simulink model "quad_sim"  (R2024b)
settings: Solver=ode4  StartTime=0.0  StopTime=qsim.StopTime  FixedStep=qsim.dt  RelTol=1e-3
PreLoadFcn:
  | if ~exist('qsim','var') || ~exist('quad','var') || ~exist('ideal','var') || ~exist('CtrlIn','var'), run(fullfile(fileparts(which('quad_sim_params')),'quad_sim_params.m')); end
values from neighbouring files (symbols this model uses):
  qsim = quad_sim_derive(qsim, quad)    [quad_scenario.m]    (also in quad_sim_params.m = quad_scenario(qsim, quad, ideal, 'hover'))
  quad = evalin('base', 'quad')    [run_quad_scenarios.m]
libraries: aerolibprivatev1p5 x1
Description:
  | Model 1: 5" quad 6-DOF plant + controller slot (Variant Subsystem "Controller", qsim.ctrl: 1 ideal, 2 board_fast, 3 board_circuit). Run quad_sim_params first.
settings Model: Creator=doubi  LastModifiedBy=doubi
settings DataIOCC: SaveOutput=off  SaveTime=off
settings DebuggingCC: AlgebraicLoopMsg=error

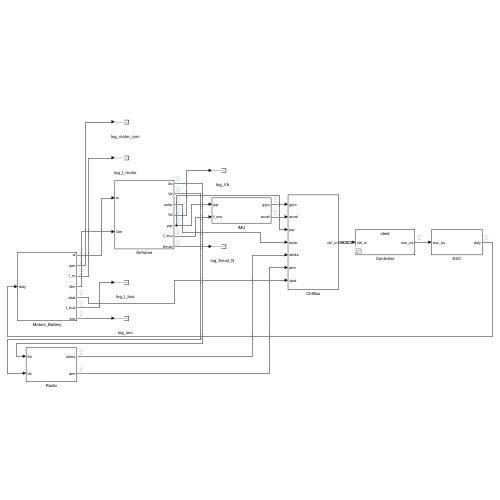
[thumbnail: Simulink's stored preview of the top-level diagram]
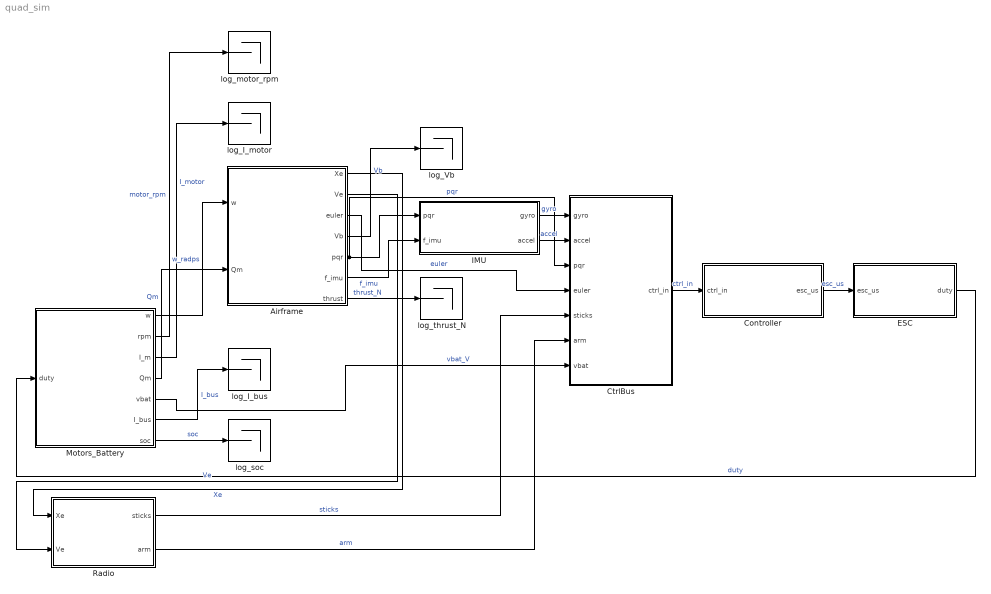
== system quad_sim ==
  Airframe : Subsystem
  Controller : Subsystem  Description=Controller slot. qsim.ctrl selects: 1 ideal (ctrl_ideal.slx), 2 board_fast, 3 board_circuit (sim/pid_board/pid_board.slx). Interface = Inport ctrl_in (bus CtrlIn), Outport esc_us [4x1] double us.  Variant=on
  CtrlBus : Subsystem
  ESC : Subsystem
  IMU : Subsystem
  Motors_Battery : Subsystem
  Radio : Subsystem
  log_I_bus : Terminator
  log_I_motor : Terminator
  log_Vb : Terminator
  log_motor_rpm : Terminator
  log_soc : Terminator
  log_thrust_N : Terminator
  wires:
  IMU/2(accel) -> CtrlBus/2(accel)  "accel"
  Motors_Battery/1(w) -> Airframe/1(w)  "w_radps"
  Motors_Battery/6(I_bus) -> log_I_bus/1  "I_bus"
  Motors_Battery/2(rpm) -> log_motor_rpm/1  "motor_rpm"
  Motors_Battery/7(soc) -> log_soc/1  "soc"
  Motors_Battery/3(I_m) -> log_I_motor/1  "I_motor"
  Motors_Battery/4(Qm) -> Airframe/2(Qm)  "Qm"
  Radio/1(sticks) -> CtrlBus/5(sticks)  "sticks"
  Motors_Battery/5(vbat) -> CtrlBus/7(vbat)  "vbat_V"
  Radio/2(arm) -> CtrlBus/6(arm)  "arm"
  Airframe/1(Xe) -> Radio/1(Xe)  "Xe"
  Airframe/2(Ve) -> Radio/2(Ve)  "Ve"
  Airframe/3(euler) -> CtrlBus/4(euler)  "euler"
  Airframe/4(Vb) -> log_Vb/1  "Vb"
  Airframe/5(pqr) -> IMU/1(pqr), CtrlBus/3(pqr)  "pqr"
  Airframe/6(f_imu) -> IMU/2(f_imu)  "f_imu"
  Airframe/7(thrust) -> log_thrust_N/1  "thrust_N"
  IMU/1(gyro) -> CtrlBus/1(gyro)  "gyro"
  CtrlBus/1(ctrl_in) -> Controller/1(ctrl_in)  "ctrl_in"
  Controller/1(esc_us) -> ESC/1(esc_us)  "esc_us"
  ESC/1(duty) -> Motors_Battery/1(duty)  "duty"

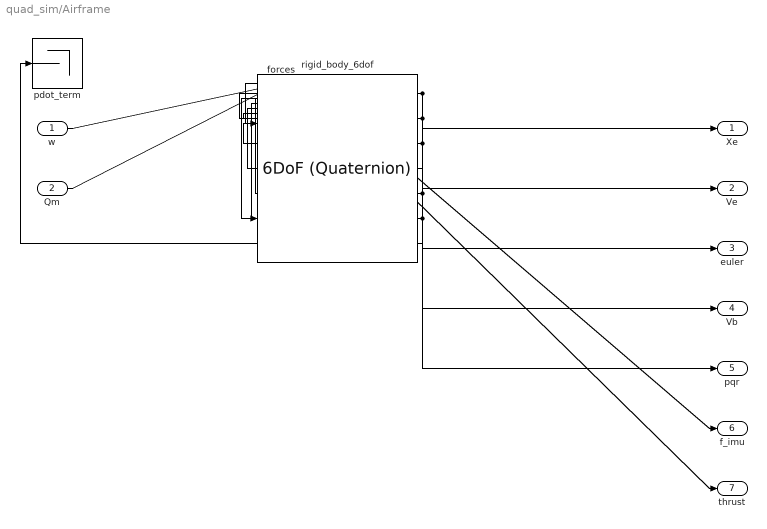
== system quad_sim/Airframe ==
  w : Inport
  Qm : Inport  Port=2
  forces : MATLAB Function  TreatAsAtomicUnit=on  mask{P=qsim.p}
  pdot_term : Terminator
  rigid_body_6dof : aerolibprivatev1p5/6DoF (Quaternion)  xme_0=qsim.init.Xe0  Vm_0=[0 0 0]  eul_0=[0 0 0]  pm_0=[0 0 0]  Mass=quad.mass.total  Inertia=quad.inertia.J  k_quat=1.0
  Xe : Outport
  Ve : Outport  Port=2
  euler : Outport  Port=3
  Vb : Outport  Port=4
  pqr : Outport  Port=5
  f_imu : Outport  Port=6
  thrust : Outport  Port=7
  wires:
  w/1 -> forces/1(w)
  Qm/1 -> forces/2(Qm)
  rigid_body_6dof/5 -> forces/3(Vb), Vb/1
  rigid_body_6dof/6 -> forces/4(wb), pqr/1
  rigid_body_6dof/4 -> forces/5(DCM)
  rigid_body_6dof/2 -> forces/6(Xe), Xe/1
  rigid_body_6dof/1 -> forces/7(Ve), Ve/1
  rigid_body_6dof/3 -> forces/8(eul), euler/1
  forces/1(F_b) -> rigid_body_6dof/1
  forces/2(M_b) -> rigid_body_6dof/2
  rigid_body_6dof/7 -> pdot_term/1
  forces/3(f_imu) -> f_imu/1
  forces/4(T) -> thrust/1

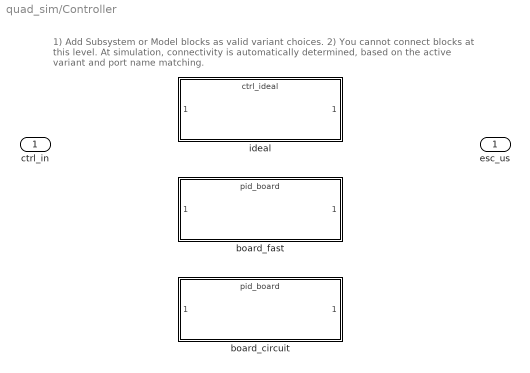
== system quad_sim/Controller ==
  note: 1) Add Subsystem or Model blocks as valid variant choices.
      | 2) You cannot connect blocks at this level. At simulation, connectivity is automatically
      | determined, based on the active variant and port name matching.
  ctrl_in : Inport
  board_circuit : ModelReference  ModelNameDialog=pid_board  ParameterArgumentNames=board_variant  ParameterArgumentValues=2  UsingDefaultArgumentValue=0  SimulationMode=Normal  VariantControl=qsim.ctrl == 3  ModelReferenceVersion=1.1
  board_fast : ModelReference  ModelNameDialog=pid_board  ParameterArgumentNames=board_variant  ParameterArgumentValues=1  UsingDefaultArgumentValue=0  SimulationMode=Normal  VariantControl=qsim.ctrl == 2  ModelReferenceVersion=1.1
  ideal : ModelReference  ModelNameDialog=ctrl_ideal  SimulationMode=Normal  VariantControl=qsim.ctrl == 1  ModelReferenceVersion=1.1
  esc_us : Outport

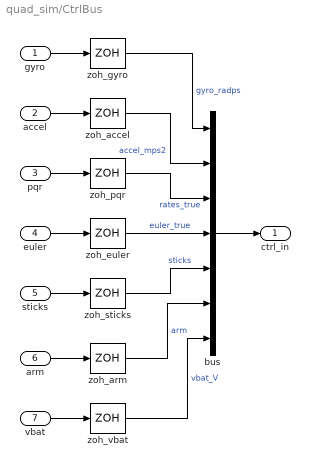
== system quad_sim/CtrlBus ==
  gyro : Inport
  accel : Inport  Port=2
  pqr : Inport  Port=3
  euler : Inport  Port=4
  sticks : Inport  Port=5
  arm : Inport  Port=6
  vbat : Inport  Port=7
  bus : BusCreator  Inputs=7  OutDataTypeStr=Bus: CtrlIn  NonVirtualBus=on
  zoh_accel : ZeroOrderHold  SampleTime=qsim.Ts_bus
  zoh_arm : ZeroOrderHold  SampleTime=qsim.Ts_bus
  zoh_euler : ZeroOrderHold  SampleTime=qsim.Ts_bus
  zoh_gyro : ZeroOrderHold  SampleTime=qsim.Ts_bus
  zoh_pqr : ZeroOrderHold  SampleTime=qsim.Ts_bus
  zoh_sticks : ZeroOrderHold  SampleTime=qsim.Ts_bus
  zoh_vbat : ZeroOrderHold  SampleTime=qsim.Ts_bus
  ctrl_in : Outport
  wires:
  sticks/1 -> zoh_sticks/1
  gyro/1 -> zoh_gyro/1
  zoh_gyro/1 -> bus/1  "gyro_radps"
  vbat/1 -> zoh_vbat/1
  arm/1 -> zoh_arm/1
  accel/1 -> zoh_accel/1
  pqr/1 -> zoh_pqr/1
  euler/1 -> zoh_euler/1
  zoh_accel/1 -> bus/2  "accel_mps2"
  zoh_pqr/1 -> bus/3  "rates_true"
  zoh_euler/1 -> bus/4  "euler_true"
  zoh_sticks/1 -> bus/5  "sticks"
  zoh_arm/1 -> bus/6  "arm"
  zoh_vbat/1 -> bus/7  "vbat_V"
  bus/1 -> ctrl_in/1

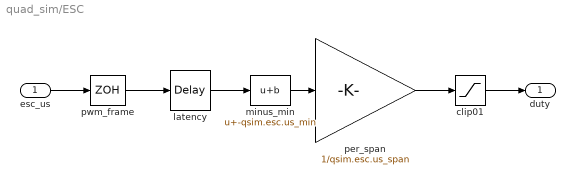
== system quad_sim/ESC ==
  esc_us : Inport
  clip01 : Saturate  UpperLimit=1  LowerLimit=0
  latency : TransportDelay  DelayTime=qsim.esc.delay  InitialOutput=qsim.esc.us0  BufferSize=4096
  minus_min : Bias  Bias=-qsim.esc.us_min  SaturateOnIntegerOverflow=off
  per_span : Gain  Gain=1/qsim.esc.us_span
  pwm_frame : ZeroOrderHold  SampleTime=qsim.esc.Ts
  duty : Outport
  wires:
  minus_min/1 -> per_span/1
  esc_us/1 -> pwm_frame/1
  pwm_frame/1 -> latency/1
  latency/1 -> minus_min/1
  per_span/1 -> clip01/1
  clip01/1 -> duty/1

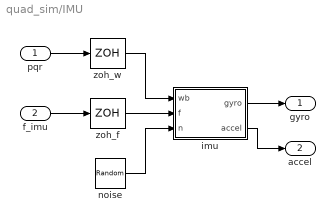
== system quad_sim/IMU ==
  pqr : Inport
  f_imu : Inport  Port=2
  imu : MATLAB Function  TreatAsAtomicUnit=on  mask{P=qsim.imu}
  noise : RandomNumber  Seed=qsim.imu.seed  SampleTime=qsim.imu.Ts
  zoh_f : ZeroOrderHold  SampleTime=qsim.imu.Ts
  zoh_w : ZeroOrderHold  SampleTime=qsim.imu.Ts
  gyro : Outport
  accel : Outport  Port=2
  wires:
  imu/2(accel) -> accel/1
  zoh_f/1 -> imu/2(f)
  pqr/1 -> zoh_w/1
  f_imu/1 -> zoh_f/1
  zoh_w/1 -> imu/1(wb)
  imu/1(gyro) -> gyro/1
  noise/1 -> imu/3(n)

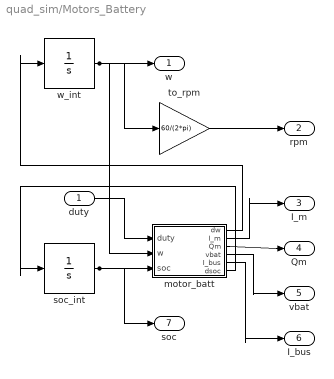
== system quad_sim/Motors_Battery ==
  duty : Inport
  motor_batt : MATLAB Function  TreatAsAtomicUnit=on  mask{P=qsim.p}
  soc_int : Integrator  InitialCondition=qsim.init.soc0  LimitOutput=on  UpperSaturationLimit=1  LowerSaturationLimit=0
  to_rpm : Gain  Gain=60/(2*pi)
  w_int : Integrator  InitialCondition=qsim.init.w0  LimitOutput=on  LowerSaturationLimit=0
  w : Outport
  rpm : Outport  Port=2
  I_m : Outport  Port=3
  Qm : Outport  Port=4
  vbat : Outport  Port=5
  I_bus : Outport  Port=6
  soc : Outport  Port=7
  wires:
  w_int/1 -> motor_batt/2(w), w/1, to_rpm/1
  to_rpm/1 -> rpm/1
  motor_batt/4(vbat) -> vbat/1
  duty/1 -> motor_batt/1(duty)
  soc_int/1 -> motor_batt/3(soc), soc/1
  motor_batt/1(dw) -> w_int/1
  motor_batt/2(I_m) -> I_m/1
  motor_batt/3(Qm) -> Qm/1
  motor_batt/5(I_bus) -> I_bus/1
  motor_batt/6(dsoc) -> soc_int/1

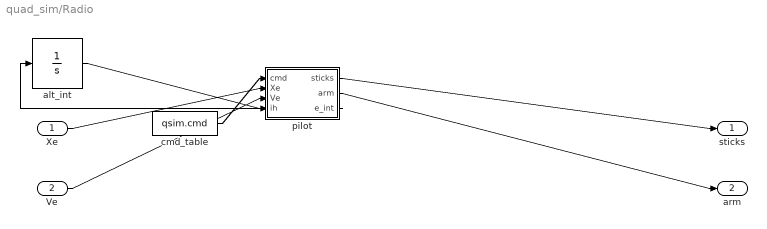
== system quad_sim/Radio ==
  Xe : Inport
  Ve : Inport  Port=2
  alt_int : Integrator
  cmd_table : FromWorkspace  VariableName=qsim.cmd  OutputAfterFinalValue=Holding final value
  pilot : MATLAB Function  TreatAsAtomicUnit=on  mask{P=qsim.pilot}
  sticks : Outport
  arm : Outport  Port=2
  wires:
  cmd_table/1 -> pilot/1(cmd)
  Xe/1 -> pilot/2(Xe)
  Ve/1 -> pilot/3(Ve)
  alt_int/1 -> pilot/4(ih)
  pilot/1(sticks) -> sticks/1
  pilot/2(arm) -> arm/1
  pilot/3(e_int) -> alt_int/1

== matlab function quad_sim/Motors_Battery/motor_batt ==
  data: duty input; dw output; w input; soc input; I_m output; Qm output; vbat output; I_bus output; dsoc output; P parameter
function [dw, I_m, Qm, vbat, I_bus, dsoc] = quad_fcn_motor_batt(duty, w, soc, P)
%QUAD_FCN_MOTOR_BATT Four DC-equivalent BLDC motors + ESCs + 4S battery.
%   Source of the "motor_batt" MATLAB Function block in quad_sim.slx
%   (quad_build_models.m copies this code into the block).
%   duty [4x1] ESC duty 0..1, w [4x1] rotor speed rad/s (>= 0), soc 0..1.
%   Model (quad_params.m, motor + battery sections):
%     ESC = ideal buck: V_m = duty*V_bus, I_in = duty*I_m (damped light,
%           so the current may go negative = active braking); duty = 0
%           means FETs off, no current.
%     motor: I_m = (V_m - w/Kv)/R   (inductance neglected, L/R << 1 ms)
%            Q_m = Kt*(I_m - I0*tanh(w/w_I0))  (no-load loss as friction)
%            J_r*dw/dt = Q_m - kQ*w^2
%     battery: V_bus = cells*OCV(soc) - R_batt*I_bus, solved in closed form
%            (no algebraic loop), I_bus = sum(duty.*I_m) + I_avionics,
%            dsoc/dt = -I_bus/capacity.
%     ESC current limit quad.esc.I_limit per channel (30 A burst).
%   Outputs: dw [4x1], I_m [4x1] A, Qm [4x1] N m (motor shaft torque, the
%   body gets -spin*Qm), vbat V, I_bus A, dsoc 1/s.

w   = w(:);
d   = min(max(duty(:), 0), 1);
on  = double(d > 0);
s   = min(max(soc, 0), 1);
E   = P.cells*interp1(P.soc_tab, P.ocv_tab, s);   % open-circuit pack voltage
emf = w/P.Kv;                                      % back-EMF, V

% V = E - Rb*(sum(on.*d.*(d*V - emf))/R + Ia)  ->  solve for V
S1 = sum(on.*d.^2)/P.R;
S2 = sum(on.*d.*emf)/P.R;
vbat = (E + P.R_batt*(S2 - P.I_av))/(1 + P.R_batt*S1);
vbat = max(vbat, 0);

I_m = on.*(d*vbat - emf)/P.R;
% ESC per-channel current limit (+-I_lim): the ESC lowers its effective duty.
% A limited channel draws P = (emf + R*I_lim)*I_lim from the bus; re-solve
% the bus voltage once with those channels as constant-power loads.
lim = double(abs(I_m) > P.I_lim);
if any(lim)
    Ilim = sign(I_m)*P.I_lim;
    Plim = sum(lim.*(emf + P.R*Ilim).*Ilim);
    u = 1 - lim;
    S1u = sum(u.*on.*d.^2)/P.R;
    S2u = sum(u.*on.*d.*emf)/P.R;
    vbat = (E + P.R_batt*(S2u - P.I_av - Plim/max(vbat, 1)))/(1 + P.R_batt*S1u);
    vbat = max(vbat, 0);
    I_m = lim.*Ilim + u.*on.*(d*vbat - emf)/P.R;
    I_bus = sum(u.*d.*I_m) + Plim/max(vbat, 1) + P.I_av;
else
    I_bus = sum(d.*I_m) + P.I_av;
end
Qm    = P.Kt*(I_m - P.I0*tanh(w/P.w_I0));
dw    = (Qm - P.kQ*w.^2)/P.J_r;
dsoc  = -I_bus/P.capacity;
end

== matlab function quad_sim/Radio/pilot ==
  data: cmd input; sticks output; Xe input; Ve input; ih input; arm output; e_int output; P parameter
function [sticks, arm, e_int] = quad_fcn_pilot(cmd, Xe, Ve, ih, P)
%QUAD_FCN_PILOT Radio commands + optional "auto pilot" on the throttle stick.
%   Source of the "pilot" MATLAB Function block in quad_sim.slx.
%   cmd = [roll pitch yaw thr arm alt_en alt_ref] from the scenario table
%   (qsim.cmd). Angle mode has no altitude loop, so to keep step tests and
%   long hovers at a constant height a simulated pilot can move the
%   throttle stick (alt_en = 1):
%       vz_cmd = sat(kh*(h_ref - h), +-vz_max)              climb-rate demand
%       thr    = thr_cmd + kvz*(vz_cmd - hdot) + ki*ih      ih = int(vz_cmd - hdot)
%   This is the PILOT, outside the controller interface (the controller just
%   sees a throttle stick). e_int feeds the external integrator (ih); it is
%   zero while alt_en = 0 or the stick is saturated (anti-windup).

cmd = cmd(:);
h = -Xe(3);  hdot = -Ve(3);          % NED -> altitude, climb rate
en = double(cmd(6) > 0.5);
vz_cmd = min(max(P.kh*(cmd(7) - h), -P.vz_max), P.vz_max);
ev = vz_cmd - hdot;
thr_raw = cmd(4) + en*(P.kvz*ev + P.ki*ih);
thr = min(max(thr_raw, 0.05), 1);
if en < 0.5, thr = min(max(cmd(4), 0), 1); end
sticks = [min(max(cmd(1:3), -1), 1); thr];
arm = double(cmd(5) > 0.5);
e_int = en*ev*double(thr == thr_raw);
end

== matlab function quad_sim/Airframe/forces ==
  data: w input; F_b output; Qm input; Vb input; wb input; DCM input; Xe input; Ve input; eul input; M_b output; f_imu output; T output; P parameter
function [F_b, M_b, f_imu, T] = quad_fcn_forces(w, Qm, Vb, wb, DCM, Xe, Ve, eul, P)
%QUAD_FCN_FORCES Body forces/moments for the 6DOF block + IMU specific force.
%   Source of the "forces" MATLAB Function block in quad_sim.slx.
%   Inputs: rotor speeds w [4x1] rad/s, motor torques Qm [4x1] N m, body
%   velocity Vb, body rates wb, DCM_be (earth->body), position Xe (NED),
%   earth velocity Ve, Euler angles eul. All forces in body FRD axes, about
%   the CG. Includes: thrust kT*w^2 at each hub (r_motor), yaw reaction
%   -spin*Qm, rotor gyroscopic moment, linear + quadratic drag, rotational
%   damping, gravity, and a simple ground (spring-damper in z, damped
%   sliding, levelling torque) for z_e > 0.
%   f_imu = specific force at the IMU location (what an accelerometer reads).

w = w(:); Qm = Qm(:); Vb = Vb(:); wb = wb(:); Xe = Xe(:); Ve = Ve(:); eul = eul(:);
T = P.kT*w.^2;                                   % N per rotor, along -z_b


% Thrust and its moment about the CG: r x [0;0;-T]
F_thr = [0; 0; -sum(T)];
M_thr = zeros(3,1);
for i = 1:4
    r = P.r_motor(:,i);
    M_thr = M_thr + [-r(2)*T(i); r(1)*T(i); 0];
end
% Yaw: stator reaction to the motor torque (includes rotor acceleration)
M_yaw = [0; 0; -sum(P.spin(:).*Qm)];
% Rotor gyroscopic moment: h = J_r*sum(spin_i*w_i)*z_b
h = [0; 0; P.J_r*sum(P.spin(:).*w)];
M_gyro = -cross(wb, h);

% Aerodynamic drag and rotational damping (no wind: airspeed = Vb)
F_drag = -P.m*P.d_lin.*Vb - 0.5*P.rho*P.CdA.*abs(Vb).*Vb;
M_damp = -P.k_rot.*wb;

% Gravity
F_grav = DCM*[0; 0; P.m*P.g];

% Ground (z_e down, ground at z_e = 0)
F_gnd_e = zeros(3,1);
M_gnd = zeros(3,1);
if Xe(3) > 0
    Fz = -(P.gnd_k*Xe(3) + P.gnd_c*Ve(3));
    Fz = min(Fz, 0);                              % ground can only push up
    F_gnd_e = [-P.gnd_cxy*Ve(1); -P.gnd_cxy*Ve(2); Fz];
    M_gnd = -P.gnd_klev*[eul(1); eul(2); 0] - P.gnd_clev*wb;
end
F_gnd = DCM*F_gnd_e;

F_b = F_thr + F_drag + F_grav + F_gnd;
M_b = M_thr + M_yaw + M_gyro + M_damp + M_gnd;

% Specific force at the IMU: non-gravitational accel + lever-arm terms
dwb = P.Jinv*(M_b - cross(wb, P.J*wb));
f_imu = (F_b - F_grav)/P.m + cross(dwb, P.r_imu) + cross(wb, cross(wb, P.r_imu));
end

== matlab function quad_sim/IMU/imu ==
  data: wb input; gyro output; f input; n input; accel output; P parameter
function [gyro, accel] = quad_fcn_imu(wb, f, n, P)
%QUAD_FCN_IMU MPU-6050 model, discrete at quad.imu.Ts (1 kHz).
%   Source of the "imu" MATLAB Function block in quad_sim.slx.
%   wb true body rates [3x1] rad/s, f specific force at the IMU [3x1] m/s^2,
%   n [6x1] unit-variance white noise (Random Number block, seeded).
%   Per axis: scale error, bias (boot-calibration residual), white noise
%   (density * sqrt(fs/2)), g-sensitivity, DLPF = 1st-order low-pass at the
%   DLPF bandwidth + an integer sample delay so the total group delay matches
%   the datasheet DLPF delay, full-scale saturation, LSB quantisation.
%   Outputs gyro rad/s, accel m/s^2 (body FRD axes; IMU axes assumed aligned).

wb = wb(:); f = f(:); n = n(:);
persistent xg xa bg ba
if isempty(xg)
    xg = wb;  xa = f;
    bg = repmat(wb, 1, 8);  ba = repmat(f, 1, 8);
end

g_raw = (1 + P.scale_g).*wb + P.bias_on*P.bias_g + P.noise_on*P.sig_g*n(1:3) ...
        + P.gsens*f/P.g;
a_raw = (1 + P.scale_a).*f + P.bias_on*P.bias_a + P.noise_on*P.sig_a*n(4:6);

xg = P.a_g*xg + (1 - P.a_g)*g_raw;
xa = P.a_a*xa + (1 - P.a_a)*a_raw;

% integer delay line (column 1 = newest)
bg = [xg, bg(:,1:7)];
ba = [xa, ba(:,1:7)];
gd = bg(:, P.nd_g + 1);
ad = ba(:, P.nd_a + 1);

gyro  = P.lsb_g*round(min(max(gd, -P.sat_g), P.sat_g)/P.lsb_g);
accel = P.lsb_a*round(min(max(ad, -P.sat_a), P.sat_a)/P.lsb_a);
end
